simulink model "Three_Phase_Two_Level_Inverter"  (R2021a)
settings: Solver=FixedStepDiscrete  StartTime=0.0  StopTime=1  FixedStep=Simulation.StepSize  RelTol=1e-3
InitFcn:
  | Simulation.StepSize = 1e-6;
  | 
  | Simulation.Inverter.P = 10e3;
  | Simulation.Inverter.Vdc = 700;
  | Simulation.Inverter.Vo = 400;%ph-ph
  | Simulation.Inverter.fo = 50;
  | 
  | Simulation.Invertion.Params.L1 = 1e-3;
  | Simulation.Invertion.Params.C1 = 100e-6;
  | 
  | Simulation.Invertion.Control.Ts = 1e-4;%1/fs
  | Simulation.Invertion.Control.fs = 10e3;%10K
  | Simulation.Invertion.Control.VoltPI.KP = 1;
  | Simulation.Invertion.Control.VoltPI.KI = 1*0.2*1e3;
  | Simulation.Invertion.Control.CurrPI.KP = 1;
undefined symbols (not defined in the file): DiscIntNeverNeededParam
libraries: spsabctodq0Lib x3, spsThreePhaseSeriesRLCBranchLib x2, pid_lib x2, spsThreePhaseVIMeasurementLib x2, spsdq0toabcLib x1, spsThreePhaseSeriesRLCLoadLib x1, spsOnDelayLib x1, spsPWMGenerator2LevelLib x1, spsTwoLevelConverterLib x1, spsDCVoltageSourceLib x1, spsVoltageMeasurementLib x1, spspowerguiLib x1
settings Model: Creator=45276  LastModifiedBy=45276

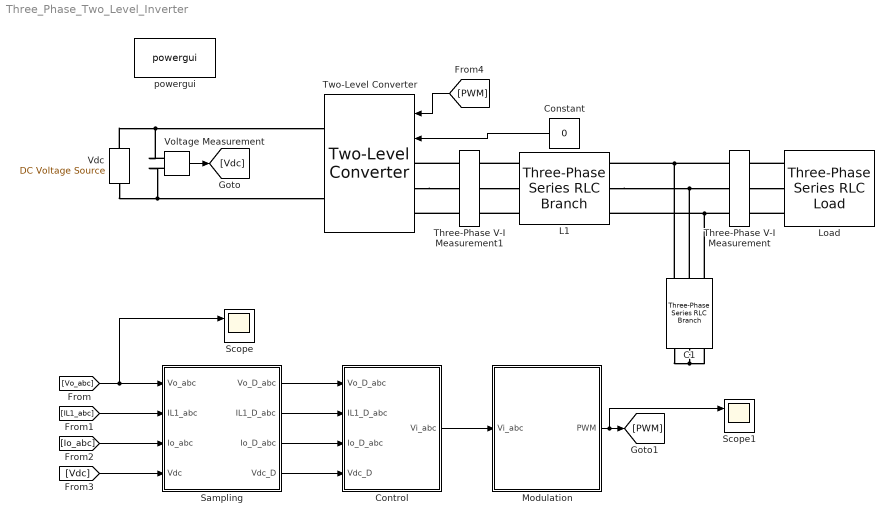
== system Three_Phase_Two_Level_Inverter ==
  C1 : spsThreePhaseSeriesRLCBranchLib/Three-Phase Series RLC Branch  LConnTagsString=A|B|C  RConnTagsString=A|B|C  BranchType=C  Resistance=1  Inductance=1e-3  Capacitance=Simulation.Invertion.Params.C1  Measurements=None
  Constant : Constant  Value=0
  Control : Subsystem
  L1 : spsThreePhaseSeriesRLCBranchLib/Three-Phase Series RLC Branch  LConnTagsString=A|B|C  RConnTagsString=A|B|C  BranchType=L  Resistance=1  Inductance=Simulation.Invertion.Params.L1  Capacitance=1e-6  Measurements=None
  Load : spsThreePhaseSeriesRLCLoadLib/Three-Phase Series RLC Load  LConnTagsString=A|B|C  Configuration=Y (grounded)  NominalVoltage=Simulation.Inverter.Vo  Vabc=[1e3 1e3 1e3]  Vabcp=[1e3 1e3 1e3]  NominalFrequency=Simulation.Inverter.fo  UnbalancedPower=off  ActivePower=Simulation.Inverter.P  InductivePower=0  CapacitivePower=0  Pabc=[10e3 9e3 11e3]  QLabc=[100 90 110]  QCabc=[100 90 110]  Pabcp=[10e3 9e3 11e3]  QLabcp=[100 90 110]  QCabcp=[100 90 110]  Measurements=None  LoadType=constant Z
  Modulation : Subsystem
  Sampling : Subsystem
  Scope : Scope  NumInputPorts=2
  Scope1 : Scope  NumInputPorts=2
  Three-Phase V-I Measurement : spsThreePhaseVIMeasurementLib/Three-Phase V-I Measurement  VoltageMeasurement=phase-to-ground  SetLabelV=on  LabelV=Vo_abc  Vpu=off  VpuLL=off  CurrentMeasurement=yes  SetLabelI=on  LabelI=Io_abc  Ipu=off  Pbase=100e6  Vbase=500e3  OutputType=Complex  PhasorSimulation=off  PSBequivalent=0
  Three-Phase V-I Measurement1 : spsThreePhaseVIMeasurementLib/Three-Phase V-I Measurement  VoltageMeasurement=no  SetLabelV=off  LabelV=Vo_abc  Vpu=off  VpuLL=off  CurrentMeasurement=yes  SetLabelI=on  LabelI=IL1_abc  Ipu=off  Pbase=100e6  Vbase=500e3  OutputType=Complex  PhasorSimulation=off  PSBequivalent=0
  Two-Level Converter : spsTwoLevelConverterLib/Two-Level Converter  ModelType=Switching devices  Ron=1e-3  Rs=1e6  Cs=inf  Vforward=[0,0]  Ron_Diode=1e-3  Rs_Diode=1e6  Cs_Diode=inf  Vf_Diode=1e-3  Rs_CurrentSource=inf
      settings: SourceProductBaseCode=PS
  Vdc : spsDCVoltageSourceLib/DC Voltage Source  Amplitude=Simulation.Inverter.Vdc  Measurements=None
  Voltage Measurement : spsVoltageMeasurementLib/Voltage Measurement  PhasorSimulation=off  OutputType=Complex  PSBequivalent=0
  powergui : spspowerguiLib/powergui  Priority=1  SimulationMode=Discrete  SampleTime=Simulation.StepSize  frequency=60  Iterations=50  frequencyindice=0  Pbase=100e6  ErrMax=1e-4  UnitsV=kV  UnitsW=MW  buscounter=0  FunctionMessages=off  echomessages=off  EnableUseOfTLC=off  CurrentSourceSwitches=off  DisableSnubberDevices=off  DisableRonSwitches=off  DisableVfSwitches=off  DisplayEquations=off  AutomaticDiscreteSolvers=off  SolverType=Tustin/Backward Euler (TBE)  Interpol=off  ExternalGateDelay=off  methode=off  Ts=100  x0status=blocks  SPID=on  SwTol=0  HookPort=off  NonlinearTolerance=1e-4  nMaxIteration=100  ContinueOnMaxIteration=off  RestoreLinks=warning  ResistiveCurrentMeasurement=off  Frange=[0:2:500]  Ylog=off  Xlog=on  ShowGrid=off  save=off  variable=ZData  structure=0  ZoomFFT=off  StartTime=0.0  cycles=1  DisplayStyle=1  fundamental=60  FreqAxis=off  MaxFrequency=1000  frequencyindicesteady=1  RmsSteady=1  display=off
  wires:
  Voltage Measurement/1 -> [Vdc]
  [Vo_abc] -> Scope/1, Sampling/1(Vo_abc)
  [IL1_abc] -> Sampling/2(IL1_abc)
  [Io_abc] -> Sampling/3(Io_abc)
  [Vdc] -> Sampling/4(Vdc)
  Sampling/1(Vo_D_abc) -> Control/1(Vo_D_abc)
  Sampling/2(IL1_D_abc) -> Control/2(IL1_D_abc)
  Sampling/3(Io_D_abc) -> Control/3(Io_D_abc)
  Sampling/4(Vdc_D) -> Control/4(Vdc_D)
  Control/1(Vi_abc) -> Modulation/1(Vi_abc)
  Modulation/1(PWM) -> Scope1/1, [PWM]
  Constant/1 -> Two-Level Converter/2
  [PWM] -> Two-Level Converter/1
  connections:
  Vdc/RConn1 -- Voltage Measurement/LConn1 -- Two-Level Converter/RConn1
  Vdc/LConn1 -- Voltage Measurement/LConn2 -- Two-Level Converter/RConn2
  L1/LConn1 -- Two-Level Converter/LConn1
  Two-Level Converter/LConn2 -- L1/LConn2
  L1/LConn3 -- Two-Level Converter/LConn3
  Load/LConn1 -- C1/LConn1 -- L1/RConn1
  L1/RConn2 -- Load/LConn2 -- C1/LConn2
  Load/LConn3 -- C1/LConn3 -- L1/RConn3
  C1/RConn1 -- C1/RConn2 -- C1/RConn3

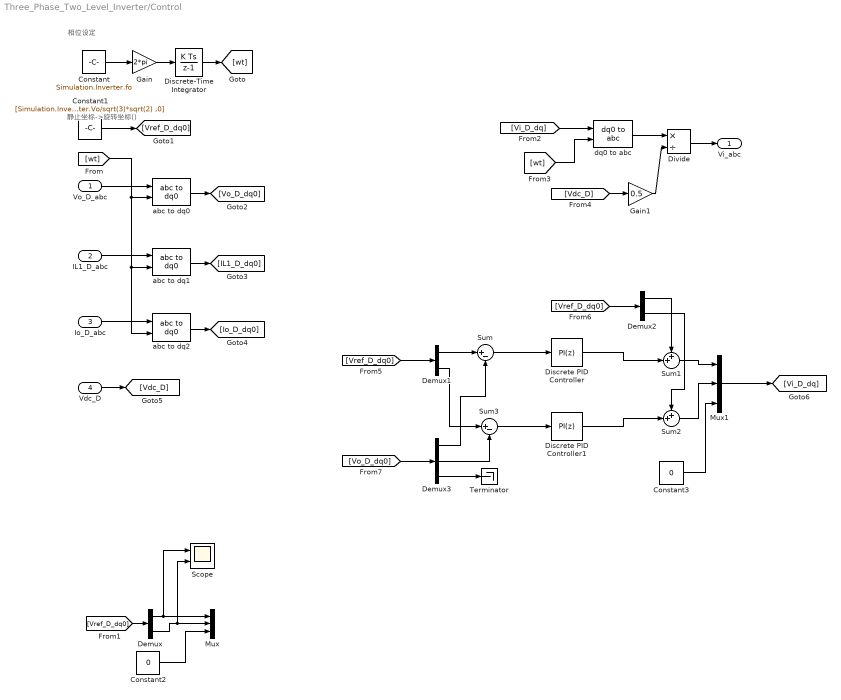
== system Three_Phase_Two_Level_Inverter/Control ==
  note: 静止坐标->旋转坐标()
  note: 相位设定
  Vo_D_abc : Inport
  IL1_D_abc : Inport  Port=2
  Io_D_abc : Inport  Port=3
  Vdc_D : Inport  Port=4
  Constant : Constant  Value=Simulation.Inverter.fo  SampleTime=Simulation.Invertion.Control.Ts
  Constant1 : Constant  Value=[Simulation.Inverter.Vo/sqrt(3)*sqrt(2) ,0]  SampleTime=Simulation.Invertion.Control.Ts
  Constant2 : Constant  Value=0
  Constant3 : Constant  Value=0
  Demux : Demux  Outputs=2
  Demux1 : Demux  Outputs=2
  Demux2 : Demux  Outputs=2
  Demux3 : Demux  Outputs=3
  Discrete PID Controller : pid_lib/PID Controller  Controller=PI  Form=Parallel  TimeDomain=Discrete-time  UseExternalTs=off  SampleTime=-1  IntegratorMethod=Forward Euler  FilterMethod=Forward Euler  ControllerParametersSource=internal  P=Simulation.Invertion.Control.VoltPI.KP  I=Simulation.Invertion.Control.VoltPI.KI  D=0  UseFilter=on  N=100  TunerSelectOption=Transfer Function Based (PID Tuner App)  InitialConditionSource=internal  InitialConditionForIntegrator=0  InitialConditionForFilter=0  DifferentiatorICPrevScaledInput=0  ExternalReset=none  TrackingMode=off  Kt=1  LimitOutput=on  SatLimitsSource=internal  UpperSaturationLimit=Simulation.Inverter.Vo/sqrt(3)*sqrt(2)*0.2  LowerSaturationLimit=-Simulation.Inverter.Vo/sqrt(3)*sqrt(2)*0.2  LinearizeAsGain=off  AntiWindupMode=none  Kb=1  POutMin=[]  POutMax=[]  IOutMin=[]  IOutMax=[]  DOutMin=[]  DOutMax=[]  NOutMin=[]  NOutMax=[]  SumOutMin=[]  SumOutMax=[]  SaturationOutMin=[]  SaturationOutMax=[]  PParamMin=[]  PParamMax=[]  IParamMin=[]  IParamMax=[]  DParamMin=[]  DParamMax=[]  NParamMin=[]  NParamMax=[]  KbParamMin=[]  KbParamMax=[]  KtParamMin=[]  KtParamMax=[]  KbOutMin=[]  KbOutMax=[]  KtOutMin=[]  KtOutMax=[]  IntegratorOutMin=[]  IntegratorOutMax=[]  FilterOutMin=[]  FilterOutMax=[]  SumI1OutMin=[]  SumI1OutMax=[]  SumI2OutMin=[]  SumI2OutMax=[]  SumI3OutMin=[]  SumI3OutMax=[]  SumI4OutMin=[]  SumI4OutMax=[]  SumDOutMin=[]  SumDOutMax=[]  DifferentiatorOutMin=[]  DifferentiatorOutMax=[]  FilterDiffOutCoefMin=[]  FilterDiffOutCoefMax=[]  ReciprocalOutMin=[]  ReciprocalOutMax=[]  SumDenOutMin=[]  SumDenOutMax=[]  SumNumOutMin=[]  SumNumOutMax=[]  DivideOutMin=[]  DivideOutMax=[]  UdiffTsProdOutMin=[]  UdiffTsProdOutMax=[]  NTsProdOutMin=[]  NTsProdOutMax=[]  UintegralTsProdOutMin=[]  UintegralTsProdOutMax=[]  UngainTsProdOutMin=[]  UngainTsProdOutMax=[]  IntegratorContinuousStateAttributes=''  IntegratorStateMustResolveToSignalObject=off  IntegratorRTWStateStorageClass=Auto  FilterContinuousStateAttributes=''  FilterStateMustResolveToSignalObject=off  FilterRTWStateStorageClass=Auto  ParallelPVariant=InternalParameters  IdealPVariant=Disabled  IVariant=InternalParameters  DVariant=Disabled  IntegratorVariant=Discrete  SatVariant=Enabled  AWVariant=Passthrough  PCopyVariant=Disabled  TRVariant=Disabled  FdbkBlocksVariant=Forward  IdealPFdbkVariant=Disabled  SatFdbkVariant=Disabled  DerivativeFilterVariant=Disabled  NVariant=Disabled  NCopyVariant=Disabled_SignalSpec  FilterICVariant=Disabled  IntegratorICVariant=InternalICs  ExternalResetVariant=Disabled  TRSumVariant=Passthrough  SumFdbkVariant=Disabled  SumVariant=Sum_PI  TsampFilterVariant=InternalTs  TsampNgainVariant=Passthrough  TsampIntegralVariant=Passthrough  ExternalSaturationOutDataTypeStr=Inherit: Same as second input
  Discrete PID Controller1 : pid_lib/PID Controller  Controller=PI  Form=Parallel  TimeDomain=Discrete-time  UseExternalTs=off  SampleTime=-1  IntegratorMethod=Forward Euler  FilterMethod=Forward Euler  ControllerParametersSource=internal  P=Simulation.Invertion.Control.VoltPI.KP  I=Simulation.Invertion.Control.VoltPI.KI  D=0  UseFilter=on  N=100  TunerSelectOption=Transfer Function Based (PID Tuner App)  InitialConditionSource=internal  InitialConditionForIntegrator=0  InitialConditionForFilter=0  DifferentiatorICPrevScaledInput=0  ExternalReset=none  TrackingMode=off  Kt=1  LimitOutput=on  SatLimitsSource=internal  UpperSaturationLimit=Simulation.Inverter.Vo/sqrt(3)*sqrt(2)*0.2  LowerSaturationLimit=-Simulation.Inverter.Vo/sqrt(3)*sqrt(2)*0.2  LinearizeAsGain=off  AntiWindupMode=none  Kb=1  POutMin=[]  POutMax=[]  IOutMin=[]  IOutMax=[]  DOutMin=[]  DOutMax=[]  NOutMin=[]  NOutMax=[]  SumOutMin=[]  SumOutMax=[]  SaturationOutMin=[]  SaturationOutMax=[]  PParamMin=[]  PParamMax=[]  IParamMin=[]  IParamMax=[]  DParamMin=[]  DParamMax=[]  NParamMin=[]  NParamMax=[]  KbParamMin=[]  KbParamMax=[]  KtParamMin=[]  KtParamMax=[]  KbOutMin=[]  KbOutMax=[]  KtOutMin=[]  KtOutMax=[]  IntegratorOutMin=[]  IntegratorOutMax=[]  FilterOutMin=[]  FilterOutMax=[]  SumI1OutMin=[]  SumI1OutMax=[]  SumI2OutMin=[]  SumI2OutMax=[]  SumI3OutMin=[]  SumI3OutMax=[]  SumI4OutMin=[]  SumI4OutMax=[]  SumDOutMin=[]  SumDOutMax=[]  DifferentiatorOutMin=[]  DifferentiatorOutMax=[]  FilterDiffOutCoefMin=[]  FilterDiffOutCoefMax=[]  ReciprocalOutMin=[]  ReciprocalOutMax=[]  SumDenOutMin=[]  SumDenOutMax=[]  SumNumOutMin=[]  SumNumOutMax=[]  DivideOutMin=[]  DivideOutMax=[]  UdiffTsProdOutMin=[]  UdiffTsProdOutMax=[]  NTsProdOutMin=[]  NTsProdOutMax=[]  UintegralTsProdOutMin=[]  UintegralTsProdOutMax=[]  UngainTsProdOutMin=[]  UngainTsProdOutMax=[]  IntegratorContinuousStateAttributes=''  IntegratorStateMustResolveToSignalObject=off  IntegratorRTWStateStorageClass=Auto  FilterContinuousStateAttributes=''  FilterStateMustResolveToSignalObject=off  FilterRTWStateStorageClass=Auto  ParallelPVariant=InternalParameters  IdealPVariant=Disabled  IVariant=InternalParameters  DVariant=Disabled  IntegratorVariant=Discrete  SatVariant=Enabled  AWVariant=Passthrough  PCopyVariant=Disabled  TRVariant=Disabled  FdbkBlocksVariant=Forward  IdealPFdbkVariant=Disabled  SatFdbkVariant=Disabled  DerivativeFilterVariant=Disabled  NVariant=Disabled  NCopyVariant=Disabled_SignalSpec  FilterICVariant=Disabled  IntegratorICVariant=InternalICs  ExternalResetVariant=Disabled  TRSumVariant=Passthrough  SumFdbkVariant=Disabled  SumVariant=Sum_PI  TsampFilterVariant=InternalTs  TsampNgainVariant=Passthrough  TsampIntegralVariant=Passthrough  ExternalSaturationOutDataTypeStr=Inherit: Same as second input
  Discrete-Time Integrator : DiscreteIntegrator  SampleTime=-1  ICPrevOutput=DiscIntNeverNeededParam  ICPrevScaledInput=DiscIntNeverNeededParam
  Divide : Product  Inputs=*/
  Gain : Gain  Gain=2*pi
  Gain1 : Gain  Gain=0.5
  Mux : Mux  Inputs=3
  Mux1 : Mux  Inputs=3
  Scope : Scope  NumInputPorts=2
  Sum : Sum  Inputs=|+-
  Sum1 : Sum  Inputs=++|
  Sum2 : Sum  Inputs=++|
  Sum3 : Sum  Inputs=|+-
  Terminator : Terminator
  abc to dq0 : spsabctodq0Lib/abc to dq0  Alignment=Aligned with phase A axis
  abc to dq1 : spsabctodq0Lib/abc to dq0  Alignment=Aligned with phase A axis
  abc to dq2 : spsabctodq0Lib/abc to dq0  Alignment=Aligned with phase A axis
  dq0 to abc : spsdq0toabcLib/dq0 to abc  Alignment=Aligned with phase A axis
  Vi_abc : Outport
  wires:
  Constant/1 -> Gain/1
  Gain/1 -> Discrete-Time Integrator/1
  Discrete-Time Integrator/1 -> [wt]
  Constant1/1 -> [Vref_D_dq0]
  IL1_D_abc/1 -> abc to dq1/1
  Io_D_abc/1 -> abc to dq2/1
  Vo_D_abc/1 -> abc to dq0/1
  abc to dq0/1 -> [Vo_D_dq0]
  abc to dq1/1 -> [IL1_D_dq0]
  abc to dq2/1 -> [Io_D_dq0]
  Vdc_D/1 -> [Vdc_D]
  [wt] -> abc to dq2/2, abc to dq1/2, abc to dq0/2
  [Vref_D_dq0] -> Demux/1
  Constant2/1 -> Mux/3
  Demux/1 -> Scope/1, Mux/1
  Demux/2 -> Scope/2, Mux/2
  [Vi_D_dq] -> dq0 to abc/1
  dq0 to abc/1 -> Divide/1
  Divide/1 -> Vi_abc/1
  [wt] -> dq0 to abc/2
  [Vdc_D] -> Gain1/1
  Gain1/1 -> Divide/2
  [Vref_D_dq0] -> Demux1/1
  [Vref_D_dq0] -> Demux2/1
  Mux1/1 -> [Vi_D_dq]
  Sum1/1 -> Mux1/1
  Sum2/1 -> Mux1/2
  [Vo_D_dq0] -> Demux3/1
  Constant3/1 -> Mux1/3
  Demux1/1 -> Sum/1
  Sum/1 -> Discrete PID Controller/1
  Demux3/1 -> Sum/2
  Demux1/2 -> Sum3/1
  Demux3/2 -> Sum3/2
  Sum3/1 -> Discrete PID Controller1/1
  Discrete PID Controller/1 -> Sum1/2
  Demux2/1 -> Sum1/1
  Demux2/2 -> Sum2/1
  Demux3/3 -> Terminator/1
  Discrete PID Controller1/1 -> Sum2/2

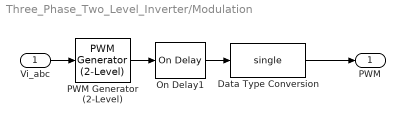
== system Three_Phase_Two_Level_Inverter/Modulation ==
  Vi_abc : Inport
  Data Type Conversion : DataTypeConversion  OutDataTypeStr=single
  On Delay1 : spsOnDelayLib/On Delay  DelayType=On delay  delay=Simulation.StepSize  ic=0  Ts=0
      settings: SourceProductBaseCode=PS
  PWM Generator (2-Level) : spsPWMGenerator2LevelLib/PWM Generator (2-Level)  ModulatorType=Three-phase bridge (6 pulses)  ModulatorMode=Unsynchronized  Fc=Simulation.Invertion.Control.fs  Pc=90  nF=27  MinMax="[ -1  1 ]"  SamplingTechnique=Natural  ModulatingSignals=off  m=0.8  Freq=60  Phase=0  Ts=0  ShowCarrierOutport=off
  PWM : Outport
  wires:
  Vi_abc/1 -> PWM Generator (2-Level)/1
  PWM Generator (2-Level)/1 -> On Delay1/1
  Data Type Conversion/1 -> PWM/1
  On Delay1/1 -> Data Type Conversion/1

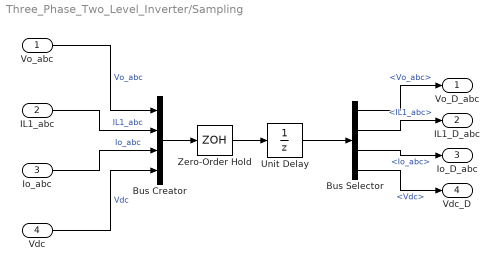
== system Three_Phase_Two_Level_Inverter/Sampling ==
  Vo_abc : Inport
  IL1_abc : Inport  Port=2
  Io_abc : Inport  Port=3
  Vdc : Inport  Port=4
  Bus Creator : BusCreator  Inputs=4
  Bus Selector : BusSelector  OutputSignals=Vo_abc,IL1_abc,Io_abc,Vdc
  Unit Delay : UnitDelay  SampleTime=-1  HasFrameUpgradeWarning=on
  Zero-Order Hold : ZeroOrderHold  SampleTime=Simulation.Invertion.Control.Ts
  Vo_D_abc : Outport
  IL1_D_abc : Outport  Port=2
  Io_D_abc : Outport  Port=3
  Vdc_D : Outport  Port=4
  wires:
  Vo_abc/1 -> Bus Creator/1  "Vo_abc"
  IL1_abc/1 -> Bus Creator/2  "IL1_abc"
  Io_abc/1 -> Bus Creator/3  "Io_abc"
  Vdc/1 -> Bus Creator/4  "Vdc"
  Bus Creator/1 -> Zero-Order Hold/1
  Zero-Order Hold/1 -> Unit Delay/1
  Unit Delay/1 -> Bus Selector/1
  Bus Selector/1 -> Vo_D_abc/1  "<Vo_abc>"
  Bus Selector/2 -> IL1_D_abc/1  "<IL1_abc>"
  Bus Selector/3 -> Io_D_abc/1  "<Io_abc>"
  Bus Selector/4 -> Vdc_D/1  "<Vdc>"
